simulink model "Airbrakes"  (R2025b)
settings: Solver=VariableStepAuto  StartTime=0.0  StopTime=10.0  RelTol=1e-3
libraries: aerolibatmos2 x1
settings Model: Creator=Bingc  LastModifiedBy=Bingc

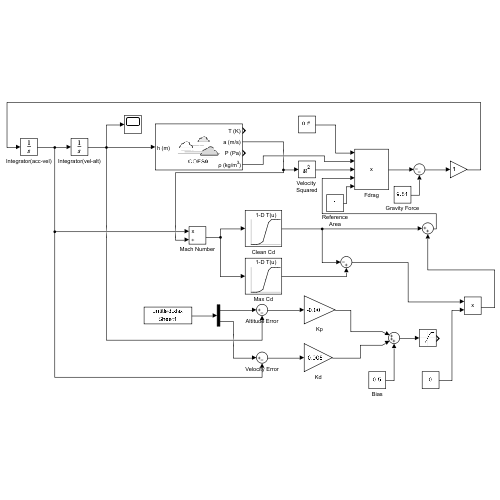
[thumbnail: Simulink's stored preview of the top-level diagram]
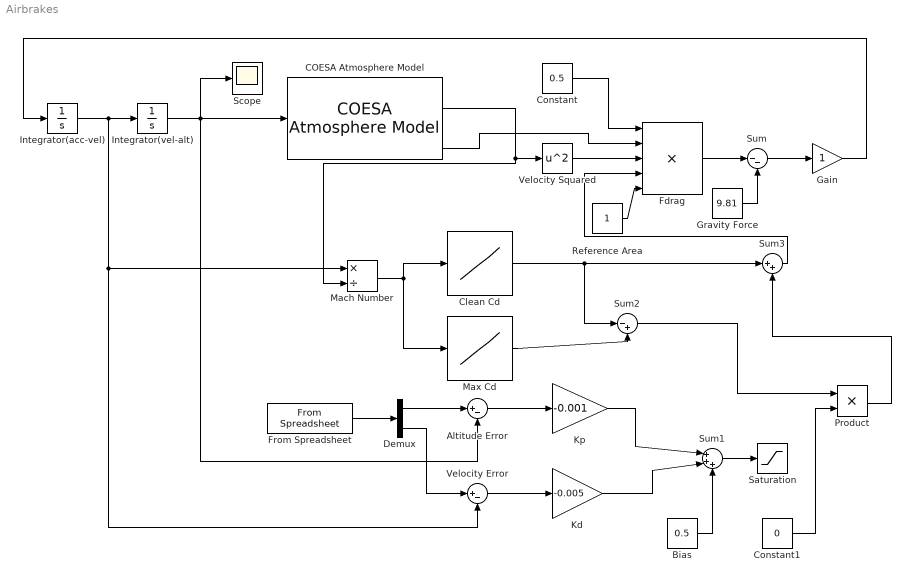
== system Airbrakes ==
  Altitude Error : Sum  Inputs=|+-
  Bias : Constant  Value=0.5
  COESA Atmosphere Model : aerolibatmos2/COESA Atmosphere Model  units=Metric (MKS)  spec=1976 COESA-extended U.S. Standard Atmosphere  model=Profile  profile_var=High temperature  profile_percent=1%  profile_alt=5 km (16404 ft)  envelope_var=High temperature  envelope_percent=1%  action=Warning
  Clean Cd : Lookup_n-D  NumberOfTableDimensions=1  BreakpointsForDimension1=[-5:5]  Table=tanh([-5:5])  InternalRulePriority=Speed  RndMeth=Simplest
  Constant : Constant  Value=0.5
  Constant1 : Constant  Value=0
  Demux : Demux  Outputs=2
  Fdrag : Product  Inputs=5
  From Spreadsheet : FromSpreadsheet
  Gain : Gain
  Gravity Force : Constant  Value=9.81
  Integrator(acc-vel) : Integrator
  Integrator(vel-alt) : Integrator
  Kd : Gain  Gain=-0.005
  Kp : Gain  Gain=-0.001
  Mach Number : Product  Inputs=*/
  Max Cd : Lookup_n-D  NumberOfTableDimensions=1  BreakpointsForDimension1=[-5:5]  Table=tanh([-5:5])  InternalRulePriority=Speed  RndMeth=Simplest
  Product : Product
  Reference Area : Constant
  Saturation : Saturate  UpperLimit=1  LowerLimit=0
  Scope : Scope
  Sum : Sum  Inputs=|--
  Sum1 : Sum  Inputs=|+++
  Sum2 : Sum  Inputs=|-+
  Sum3 : Sum  Inputs=|++
  Velocity Squared : Math  Operator=square
  Velocity Error : Sum  Inputs=|+-
  wires:
  Integrator(acc-vel)/1 -> Velocity Error/2, Mach Number/1, Integrator(vel-alt)/1
  Integrator(vel-alt)/1 -> Altitude Error/2, COESA Atmosphere Model/1, Scope/1
  COESA Atmosphere Model/2 -> Mach Number/2, Velocity Squared/1
  Constant/1 -> Fdrag/1
  COESA Atmosphere Model/4 -> Fdrag/2
  Velocity Squared/1 -> Fdrag/3
  Mach Number/1 -> Max Cd/1, Clean Cd/1
  Clean Cd/1 -> Sum2/1, Sum3/1
  Fdrag/1 -> Sum/1
  Gravity Force/1 -> Sum/2
  Sum/1 -> Gain/1
  From Spreadsheet/1 -> Demux/1
  Demux/1 -> Altitude Error/1
  Demux/2 -> Velocity Error/1
  Altitude Error/1 -> Kp/1
  Velocity Error/1 -> Kd/1
  Kp/1 -> Sum1/1
  Kd/1 -> Sum1/2
  Bias/1 -> Sum1/3
  Sum1/1 -> Saturation/1
  Max Cd/1 -> Sum2/2
  Sum2/1 -> Product/1
  Product/1 -> Sum3/2
  Gain/1 -> Integrator(acc-vel)/1
  Sum3/1 -> Fdrag/4
  Reference Area/1 -> Fdrag/5
  Constant1/1 -> Product/2
